simulink model "single_phase_ttype_inverter"  (R2026a)
settings: Solver=ode23tb  StopTime=simlength  FixedStep=tc  MaxStep=glb_time.tc
values from neighbouring files (symbols this model uses):
  afe_ctrl = param.afe.ctrl    [init_model.m]
  afe_pwm_phase_shift_mod1 = param.afe.behav.pwm_phase_shift_mod1    [init_model.m]
  DThs_init = param.thermal.DThs_init    [init_model.m]
  filters = param.ctrl.filters    [init_model.m]
  frt_data = param.frt.data    [init_model.m]
  glb_time = param.glb_time    [init_model.m]
  grid_emu = param.grid.emu    [init_model.m]
  kepsilon = param.spinv.kepsilon    [init_model.m]
  kp_align = param.ctrl.kp_align    [init_model.m]
  lim_down_align = param.ctrl.lim_down_align    [init_model.m]
  lim_up_align = param.ctrl.lim_up_align    [init_model.m]
  mavarage_filter_frequency_base_order = param.ctrl.mavarage_filter_frequency_base_order    [init_model.m]
  omega_set = param.spinv.omega_set    [init_model.m]
  single_phase_inverter_ctrl = param.spinv.ctrl    [init_model.m]
  Tambient = param.thermal.Tambient    [init_model.m]
  time_aux_power_supply_fault = param.sim.time_aux_power_supply_fault    [init_model.m]
  time_step_ref_1 = param.spinv.ref.time_step_ref_1    [init_model.m]
  time_step_ref_2 = param.spinv.ref.time_step_ref_2    [init_model.m]
  time_step_ref_3 = param.spinv.ref.time_step_ref_3    [init_model.m]
undefined symbols (not defined in the file or in its folder): delta_fht1, hwdata, ki_align, Ld_fht1, magnitude, omega_fht1, ts_inv, Vac_FS, Vdc_nom, Xbez
libraries: fl_lib x61, nesl_utility x39, moving_average_filter x11, moving_average_filter_cc x8, discrete_time_low_pass_filter x4, sl_discontinuities x3, single_phase_transformer_lib x3, linear_double_integrator_observer_ccaller x2, phase_shift_filter_ccaller x2, threephase_inductor_lib x1, dclink_for_two_levels x1, three_phase_pwm_modulator x1
(part 1 of 9)
settings Model: SimulationMode=accelerator  Creator=LTNBDA  LastModifiedBy=dbagn
settings SolverCC: ZeroCrossControl=EnableAll  ZeroCrossAlgorithm=Adaptive  SolverResetMethod=Robust
settings DataIOCC: MaxDataPoints=1  SignalLoggingSaveFormat=ModelDataLogs
settings OptimizationCC: InitFltsAndDblsToZero=on  EfficientMapNaN2IntZero=off
settings DebuggingCC: SaveWithParameterizedLinksMsg=none  UnderspecifiedInitializationDetection=Classic  SignalResolutionControl=TryResolveAllWithWarning  IgnoredZcDiagnostic=none  MultiTaskDSMMsg=warning  MultiTaskCondExecSysMsg=none  MultiTaskRateTransMsg=warning
settings HardwareCC: ProdBitPerLong=64.0  ProdHWDeviceType=Generic->64-bit Embedded Processor (LP64)  TargetBitPerPointer=64.0  TargetBitPerSizeT=64.0  TargetBitPerPtrDiffT=64.0  TargetLongLongMode=on  TargetIntDivRoundTo=Zero  TargetEndianess=LittleEndian  TargetWordSize=64.0  TargetHWDeviceType=MATLAB Host  ProdEqTarget=off
settings SFSimCC: SimCustomHeaderCode=|
  | #include "rpi.h"
  | #include "rpi_simulink.h"
  | #include "mavgflt.h"
  | #include "mavgflt_simulink.h"
  | #include "mavgflts.h"
  | #include "mavgflts_simulink.h"
  | #include "dsmavgflt.h"
  | #include "dsmavgflt_simulink.h"
  | #include "bemf_obsv.h"
  | #include "bemf_obsv_simulink.h"
  | #include "bemf_obsv_load_est.h"
  | #include "bemf_obsv_load_est_simulink.h"
  | #include "dqvector_pi.h"
  | #include "dqvector_pi_simulink.h"
  | #include "sv_pwm_simulink.h"
  | #include "sv_pwm.h"
  | #include "first_harmonic_tracker.h"
  | #include "first_harmonic_tracker_simulink.h"
  | #include "dqpll_thyr.h"
  | #include "dqpll_thyr_simulink.h"
  | #include "dqpll_grid.h"
  | #include "dqpll_grid_simulink.h"
  | #include "phase_shift_flt_simulink.h"
  | #include "phase_shift_flt.h"
  | #include "sogi_flt_simulink.h"
  | #include "sogi_flt.h"
  | #include "linear_double_integrator_observer_simulink.h"
  | #include "linear_double_integrator_observer.h"
settings SFSimCC: SimUserSources=|
  | "rpi.c"
  | "rpi_simulink.c"
  | "mavgflt_simulink.c"
  | "mavgflt.c"
  | "mavgflts_simulink.c"
  | "mavgflts.c"
  | "dsmavgflt_simulink.c"
  | "dsmavgflt.c"
  | "bemf_obsv_simulink.c"
  | "bemf_obsv.c"
  | "bemf_obsv_load_est_simulink.c"
  | "bemf_obsv_load_est.c"
  | "dqvector_pi.c"
  | "dqvector_pi_simulink.c"
  | "sv_pwm_simulink.c"
  | "sv_pwm.c"
  | "first_harmonic_tracker_simulink.c"
  | "first_harmonic_tracker.c"
  | "dqpll_thyr_simulink.c"
  | "dqpll_thyr.c"
  | "dqpll_grid_simulink.c"
  | "dqpll_grid.c"
  | "phase_shift_flt_simulink.c"
  | "phase_shift_flt.c"
  | "sogi_flt_simulink.c"
  | "sogi_flt.c"
  | "linear_double_integrator_observer_simulink.c"
  | "linear_double_integrator_observer.c"
settings SFSimCC: SimUserIncludeDirs=|
  | include
  | src
settings CodeAppCC: MaxIdLength=128.0
settings GRTTargetCC: CombineOutputUpdateFcns=off  GRTInterface=on
settings SimscapeCC: SimscapeNormalizeSystem=off  SimscapeNominalValues="[{\"value\":\"1\",\"unit\":\"A\"},{\"value\":\"1\",\"unit\":\"bar\"},{\"value\":\"1\",\"unit\":\"cm^2\"},{\"value\":\"1\",\"unit\":\"cm^3/s\"},{\"value\":\"1\",\"unit\":\"kJ/kg\"},{\"value\":\"1\",\"unit\":\"kW\"},{\"value\":\"1\",\"unit\":\"l\"},{\"value\":\"1\",\"unit\":\"N\"},{\"value\":\"1\",\"unit\":\"N*m\"},{\"value\":\"1\",\"unit\":\"V\"}]"  SimscapeLogType=none  SimscapeLogDataHistory=5000.0

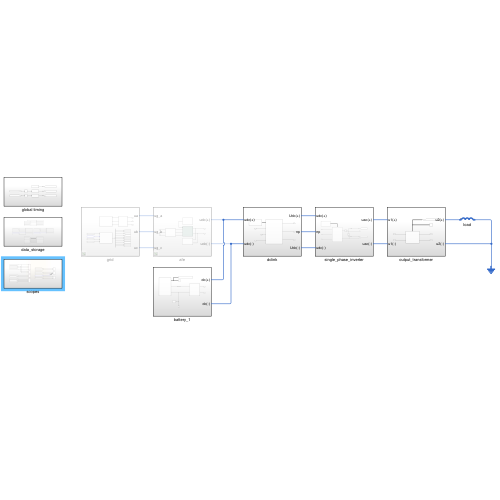
[thumbnail: Simulink's stored preview of the top-level diagram]
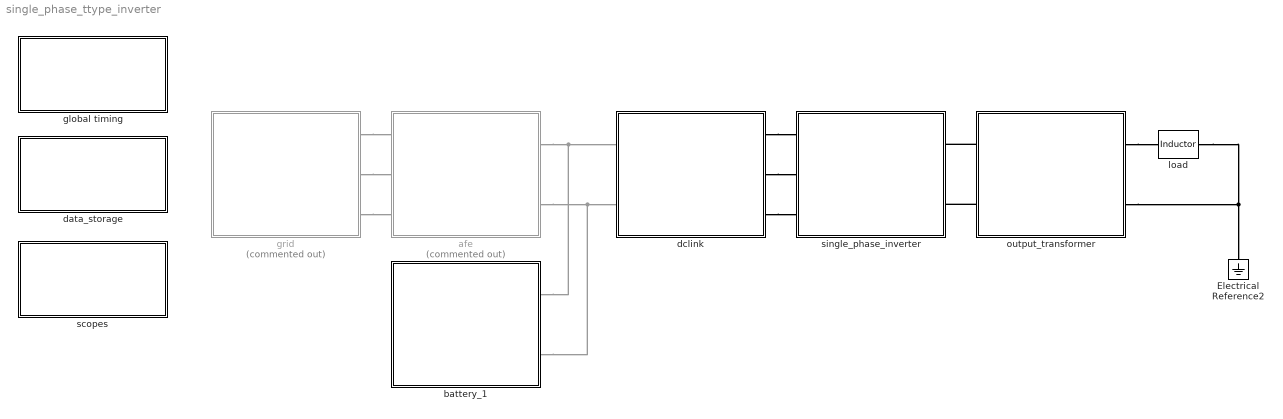
== system single_phase_ttype_inverter ==
  Electrical Reference2 : fl_lib/Electrical/Electrical Elements/Electrical Reference
  afe : Subsystem  Commented=on
  battery_1 : Subsystem
  data_storage : Subsystem
  dclink : Subsystem
  global timing : Subsystem
  grid : Subsystem  Commented=on
  load : fl_lib/Electrical/Electrical Elements/Inductor  l=lload H  r=rload Ohm  g=1e-9 1/Ohm  i_specify=off  i_priority=None  i=0 A  i_nominal_specify=off  i_nominal_value=1  i_nominal_unit=A  v_specify=off  v_priority=None  v=0 V  v_nominal_specify=off  v_nominal_value=1  v_nominal_unit=V  i_L_specify=off  i_L_priority=High  i_L=0 A  i_L_nominal_specify=off  i_L_nominal_value=1  i_L_nominal_unit=A
  output_transformer : Subsystem
  scopes : Subsystem
  single_phase_inverter : Subsystem
  connections:
  output_transformer/LConn1 -- single_phase_inverter/RConn1
  output_transformer/LConn2 -- single_phase_inverter/RConn2
  load/RConn1 -- output_transformer/RConn2 -- Electrical Reference2/LConn1
  output_transformer/RConn1 -- load/LConn1
  dclink/RConn1 -- single_phase_inverter/LConn1
  dclink/RConn2 -- single_phase_inverter/LConn2
  dclink/RConn3 -- single_phase_inverter/LConn3
  afe/RConn2 -- battery_1/RConn2 -- dclink/LConn2
  afe/RConn1 -- battery_1/RConn1 -- dclink/LConn1
  grid/RConn1 -- afe/LConn1
  grid/RConn2 -- afe/LConn2
  grid/RConn3 -- afe/LConn3

== system single_phase_ttype_inverter/afe ==
  AFE_control : Subsystem
  LCL_filter : Subsystem
  afe : Subsystem
  brake : Subsystem
  ug_a : PMIOPort  Side=Left
  udc(+) : PMIOPort  Port=2  Side=Right
  ug_b : PMIOPort  Port=3  Side=Left
  udc(-) : PMIOPort  Port=4  Side=Right
  ug_c : PMIOPort  Port=5  Side=Left
  wires:
  AFE_control/1(dabc_out) -> afe/1(dabc)
  connections:
  brake/LConn2 -- udc(-)/RConn1 -- afe/RConn2
  brake/LConn1 -- udc(+)/RConn1 -- afe/RConn1
  LCL_filter/LConn1 -- afe/LConn1
  LCL_filter/LConn2 -- afe/LConn2
  LCL_filter/LConn3 -- afe/LConn3
  ug_a/RConn1 -- LCL_filter/RConn1
  ug_b/RConn1 -- LCL_filter/RConn2
  ug_c/RConn1 -- LCL_filter/RConn3

== system single_phase_ttype_inverter/battery_1 ==
  Electrical Reference : fl_lib/Electrical/Electrical Elements/Electrical Reference
  Inductor : fl_lib/Electrical/Electrical Elements/Inductor  l=1e-3 H  r=0 Ohm  g=1e-9 1/Ohm  i_specify=off  i_priority=None  i=0 A  i_nominal_specify=off  i_nominal_value=1  i_nominal_unit=A  v_specify=off  v_priority=None  v=0 V  v_nominal_specify=off  v_nominal_value=1  v_nominal_unit=V  i_L_specify=off  i_L_priority=High  i_L=0 A  i_L_nominal_specify=off  i_L_nominal_value=1  i_L_nominal_unit=A
  Solver Configuration : nesl_utility/Solver Configuration  PhysicalDomain=network_engine_domain  SubClassName=solver  LeftPortType=input  RightPortType=generic  Tones=[]  Harmonics=[]  SimulateNoise=off  Profile=off  UseLocalSampling=off  EnableSwitchedLinearOptims=on  FrequencyDomain=off  UseCCode=off  RelTol=0.001  AbsTol=0.001  MinStep=1e-09  ToWorkspace=off  RevertToSquareIcSolve=off  NumHomotopyIterations=100  PhasorMode=off  PhasorModeNumHarmonics=1  ConsistencySolver=NEWTON_FTOL  CanonicalOrdering=UNORDERED  OptimizeIntermediates=UNOPTIMIZED  IndexReductionMethod=DerivativeReplacement  DoDC=on  ResidualTolerance=1e-3  ConsistencyTolSource=GLOBAL  ConsistencyAbsTol=0.001  ConsistencyRelTol=0.001  ConsistencyTolFactor=0.001  UseLocalSolver=on  LocalSolverChoice=NE_BACKWARD_EULER_ADVANCER  ResolveIndetEquations=on  FunctionEvalNumThread=1  LocalSolverSampleTime=glb_time.tc  DoFixedCost=on  MaxNonlinIter=nonlinear_iterations  MaxModeIter=2  ComputeImpulses=off  ImpulseIterations=2  LinearAlgebra=auto  LinearAlgebraNumThread=0  EquationFormulation=NE_TIME_EF  DelaysMemoryBudget=1024  AutomaticFiltering=on  FilteringTimeConstant=0.001  PartitionStorageMethod=AS_NEEDED  PartitionMemoryBudget=1024  PartitionMethod=ROBUST  MultibodyUseLocalSolver=off  MultibodyLocalSolverChoice=ODE1  MultibodyLocalSolverSampleTime=0.001
  To Workspace14 : ToWorkspace  VariableName=battery_1_data_sim  SampleTime=glb_time.tc
      settings: MaxDataPoints=glb_time.Nc  Decimation=glb_time.decimation_tc
  lithium ion battery : Scope
      settings: ActiveDisplayYMinimum=-808.27997881012811  ActiveDisplayYMaximum=1287.7546757937268  DataLoggingVariableName=ScopeData3
  lithium_ion_battery : lithium_ion_battery/lithium_ion_battery  Q=lithium_ion_battery_1.Q  number_of_cells=lithium_ion_battery_1.number_of_cells  E_1=lithium_ion_battery_1.E_1  E0=lithium_ion_battery_1.E0  E1=lithium_ion_battery_1.E1  E2=lithium_ion_battery_1.E2  E3=lithium_ion_battery_1.E3  Elog=lithium_ion_battery_1.Elog  R0=lithium_ion_battery_1.R0  R1=lithium_ion_battery_1.R1  C1=lithium_ion_battery_1.C1  M=lithium_ion_battery_1.M  alpha=lithium_ion_battery_1.alpha  soc_init=lithium_ion_battery_1.soc_init  ts_battery=glb_time.ts_dab  q1Kalman=lithium_ion_battery_1.q1Kalman  q2Kalman=lithium_ion_battery_1.q2Kalman  q3Kalman=lithium_ion_battery_1.q3Kalman  rKalman=lithium_ion_battery_1.rKalman  tc=glb_time.tc  enable_white_noise_m=0
  single_phase_ui_measure : Subsystem
  dc(+) : PMIOPort  Side=Right
  dc(-) : PMIOPort  Port=2  Side=Right
  wires:
  lithium_ion_battery/1 -> To Workspace14/1, lithium ion battery/1
  connections:
  lithium_ion_battery/RConn2 -- single_phase_ui_measure/LConn2 -- Solver Configuration/RConn1 -- Electrical Reference/LConn1
  single_phase_ui_measure/RConn1 -- dc(+)/RConn1
  Inductor/LConn1 -- lithium_ion_battery/RConn1
  dc(-)/RConn1 -- single_phase_ui_measure/RConn2
  single_phase_ui_measure/LConn1 -- Inductor/RConn1

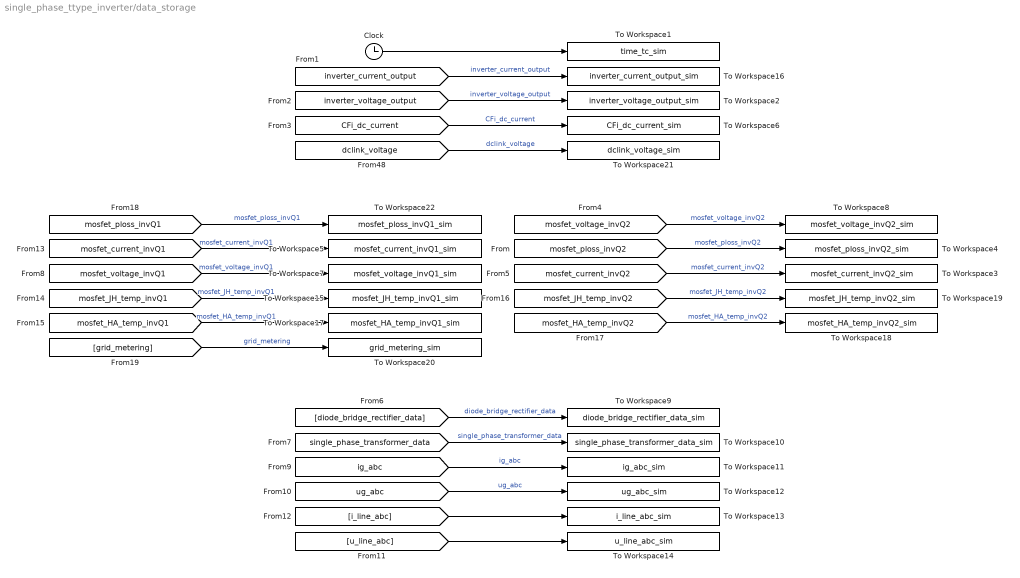
== system single_phase_ttype_inverter/data_storage ==
  Clock : Clock
  To Workspace1 : ToWorkspace  VariableName=time_tc_sim  SampleTime=glb_time.tc
      settings: MaxDataPoints=glb_time.Nc  Decimation=glb_time.decimation_tc
  To Workspace10 : ToWorkspace  VariableName=single_phase_transformer_data_sim  SampleTime=glb_time.tc
      settings: MaxDataPoints=glb_time.Nc  Decimation=glb_time.decimation_tc
  To Workspace11 : ToWorkspace  VariableName=ig_abc_sim  SampleTime=glb_time.tc
      settings: MaxDataPoints=glb_time.Nc  Decimation=glb_time.decimation_tc
  To Workspace12 : ToWorkspace  VariableName=ug_abc_sim  SampleTime=glb_time.tc
      settings: MaxDataPoints=glb_time.Nc  Decimation=glb_time.decimation_tc
  To Workspace13 : ToWorkspace  VariableName=i_line_abc_sim  SampleTime=glb_time.tc
      settings: MaxDataPoints=glb_time.Nc  Decimation=glb_time.decimation_tc
  To Workspace14 : ToWorkspace  VariableName=u_line_abc_sim  SampleTime=glb_time.tc
      settings: MaxDataPoints=glb_time.Nc  Decimation=glb_time.decimation_tc
  To Workspace15 : ToWorkspace  VariableName=mosfet_JH_temp_invQ1_sim  SampleTime=glb_time.tc
      settings: MaxDataPoints=glb_time.Nc  Decimation=glb_time.decimation_tc
  To Workspace16 : ToWorkspace  VariableName=inverter_current_output_sim  SampleTime=glb_time.tc
      settings: MaxDataPoints=glb_time.Nc  Decimation=glb_time.decimation_tc
  To Workspace17 : ToWorkspace  VariableName=mosfet_HA_temp_invQ1_sim  SampleTime=glb_time.tc
      settings: MaxDataPoints=glb_time.Nc  Decimation=glb_time.decimation_tc
  To Workspace18 : ToWorkspace  VariableName=mosfet_HA_temp_invQ2_sim  SampleTime=glb_time.tc
      settings: MaxDataPoints=glb_time.Nc  Decimation=glb_time.decimation_tc
  To Workspace19 : ToWorkspace  VariableName=mosfet_JH_temp_invQ2_sim  SampleTime=glb_time.tc
      settings: MaxDataPoints=glb_time.Nc  Decimation=glb_time.decimation_tc
  To Workspace2 : ToWorkspace  VariableName=inverter_voltage_output_sim  SampleTime=glb_time.tc
      settings: MaxDataPoints=glb_time.Nc  Decimation=glb_time.decimation_tc
  To Workspace20 : ToWorkspace  VariableName=grid_metering_sim  SampleTime=glb_time.tc
      settings: MaxDataPoints=glb_time.Nc  Decimation=glb_time.decimation_tc
  To Workspace21 : ToWorkspace  VariableName=dclink_voltage_sim  SampleTime=glb_time.tc
      settings: MaxDataPoints=glb_time.Nc  Decimation=glb_time.decimation_tc
  To Workspace22 : ToWorkspace  VariableName=mosfet_ploss_invQ1_sim  SampleTime=glb_time.tc
      settings: MaxDataPoints=glb_time.Nc  Decimation=glb_time.decimation_tc
  To Workspace3 : ToWorkspace  VariableName=mosfet_current_invQ2_sim  SampleTime=glb_time.tc
      settings: MaxDataPoints=glb_time.Nc  Decimation=glb_time.decimation_tc
  To Workspace4 : ToWorkspace  VariableName=mosfet_ploss_invQ2_sim  SampleTime=glb_time.tc
      settings: MaxDataPoints=glb_time.Nc  Decimation=glb_time.decimation_tc
  To Workspace5 : ToWorkspace  VariableName=mosfet_current_invQ1_sim  SampleTime=glb_time.tc
      settings: MaxDataPoints=glb_time.Nc  Decimation=glb_time.decimation_tc
  To Workspace6 : ToWorkspace  VariableName=CFi_dc_current_sim  SampleTime=glb_time.tc
      settings: MaxDataPoints=glb_time.Nc  Decimation=glb_time.decimation_tc
  To Workspace7 : ToWorkspace  VariableName=mosfet_voltage_invQ1_sim  SampleTime=glb_time.tc
      settings: MaxDataPoints=glb_time.Nc  Decimation=glb_time.decimation_tc
  To Workspace8 : ToWorkspace  VariableName=mosfet_voltage_invQ2_sim  SampleTime=glb_time.tc
      settings: MaxDataPoints=glb_time.Nc  Decimation=glb_time.decimation_tc
  To Workspace9 : ToWorkspace  VariableName=diode_bridge_rectifier_data_sim  SampleTime=glb_time.tc
      settings: MaxDataPoints=glb_time.Nc  Decimation=glb_time.decimation_tc
  wires:
  Clock/1 -> To Workspace1/1
  [inverter_current_output] -> To Workspace16/1  "inverter_current_output"
  [inverter_voltage_output] -> To Workspace2/1  "inverter_voltage_output"
  [CFi_dc_current] -> To Workspace6/1  "CFi_dc_current"
  [mosfet_ploss_invQ1] -> To Workspace22/1  "mosfet_ploss_invQ1"
  [dclink_voltage] -> To Workspace21/1  "dclink_voltage"
  [mosfet_current_invQ1] -> To Workspace5/1  "mosfet_current_invQ1"
  [mosfet_current_invQ2] -> To Workspace3/1  "mosfet_current_invQ2"
  [mosfet_ploss_invQ2] -> To Workspace4/1  "mosfet_ploss_invQ2"
  [mosfet_voltage_invQ1] -> To Workspace7/1  "mosfet_voltage_invQ1"
  [mosfet_voltage_invQ2] -> To Workspace8/1  "mosfet_voltage_invQ2"
  [diode_bridge_rectifier_data] -> To Workspace9/1  "diode_bridge_rectifier_data"
  [single_phase_transformer_data] -> To Workspace10/1  "single_phase_transformer_data"
  [ig_abc] -> To Workspace11/1  "ig_abc"
  [ug_abc] -> To Workspace12/1  "ug_abc"
  [i_line_abc] -> To Workspace13/1
  [u_line_abc] -> To Workspace14/1
  [mosfet_JH_temp_invQ1] -> To Workspace15/1  "mosfet_JH_temp_invQ1"
  [mosfet_HA_temp_invQ1] -> To Workspace17/1  "mosfet_HA_temp_invQ1"
  [mosfet_JH_temp_invQ2] -> To Workspace19/1  "mosfet_JH_temp_invQ2"
  [mosfet_HA_temp_invQ2] -> To Workspace18/1  "mosfet_HA_temp_invQ2"
  [grid_metering] -> To Workspace20/1  "grid_metering"

== system single_phase_ttype_inverter/dclink ==
  Open Circuit : fl_lib/Electrical/Electrical Elements/Open Circuit  v_specify=off  v_priority=None  v=0 V  v_nominal_specify=off  v_nominal_value=1  v_nominal_unit=V
  dclink : dclink_for_three_levels/dclink  Cdc1_m=hwdata.single_phase_inverter.CFi1  Cdc2_m=hwdata.single_phase_inverter.CFi2  Rudc_measure=107e3  Vdc_scale=hwdata.single_phase_inverter.udc_nom  Vdc1_m_init=hwdata.single_phase_inverter.udc_nom/2  Vdc2_m_init=hwdata.single_phase_inverter.udc_nom/2
  references : Subsystem
  Udc(+) : PMIOPort  Side=Right
  np : PMIOPort  Port=2  Side=Right
  Udc(-) : PMIOPort  Port=3  Side=Right
  udc(+) : PMIOPort  Port=4  Side=Left
  udc(-) : PMIOPort  Port=5  Side=Left
  wires:
  dclink/1 -> references/1(m)
  connections:
  Open Circuit/LConn1 -- dclink/RConn2
  udc(+)/RConn1 -- dclink/RConn1
  udc(-)/RConn1 -- dclink/RConn3
  Udc(+)/RConn1 -- dclink/LConn1
  Udc(-)/RConn1 -- dclink/LConn3
  dclink/LConn2 -- np/RConn1

== system single_phase_ttype_inverter/global timing ==
  Unit Delay : UnitDelay  SampleTime=glb_time.tc
  Unit Delay1 : UnitDelay  SampleTime=glb_time.tc
  time_afe1 : Subsystem  mask{k=1}
      mask prompts: k "Time Gain"
      mask Display:
      | disp('time-gen');
      | port_label('input', 1, 'crt');
      | port_label('output', 1, 'tout');
  time_afe2 : Subsystem  mask{k=1}
      mask prompts: k "Time Gain"
      mask Display:
      | disp('time-gen');
      | port_label('input', 1, 'crt');
      | port_label('output', 1, 'tout');
  time_afe3 : Subsystem  mask{k=1}
      mask prompts: k "Time Gain"
      mask Display:
      | disp('time-gen');
      | port_label('output', 1, 'tout');
  tag scope: local_time_afe=global, local_time_inverter=global, time_master=global
  wires:
  time_afe1/1(Out1) -> [local_time_afe]
  time_afe3/1(Out1) -> [time_master]
  [local_time_corr_afe] -> Unit Delay/1
  Unit Delay/1 -> time_afe1/1(correction_time)
  Unit Delay1/1 -> time_afe2/1(correction_time)
  [local_time_corr_inv] -> Unit Delay1/1
  time_afe2/1(Out1) -> [local_time_inverter]

== system single_phase_ttype_inverter/grid ==
  Bus Selector : BusSelector  OutputSignals=Q1p,Q1n,P1n,P1p,U1n,U1p,i_act_1n,i_react_1n,i_act_1p,i_react_1p
  To Workspace1 : ToWorkspace  VariableName=i_react_1n  SampleTime=glb_time.ts_afe
      settings: MaxDataPoints=glb_time.Ns_afe
  To Workspace2 : ToWorkspace  VariableName=i_react_1p  SampleTime=glb_time.ts_afe
      settings: MaxDataPoints=glb_time.Ns_afe
  To Workspace3 : ToWorkspace  VariableName=i_act_1n  SampleTime=glb_time.ts_afe
      settings: MaxDataPoints=glb_time.Ns_afe
  To Workspace4 : ToWorkspace  VariableName=i_act_1p  SampleTime=glb_time.ts_afe
      settings: MaxDataPoints=glb_time.Ns_afe
  To Workspace5 : ToWorkspace  VariableName=u1p  SampleTime=glb_time.ts_afe
      settings: MaxDataPoints=glb_time.Ns_afe
  To Workspace6 : ToWorkspace  VariableName=u1n  SampleTime=glb_time.ts_afe
      settings: MaxDataPoints=glb_time.Ns_afe
  grid_emulator : Subsystem
  power meter iec : power_meter_iec/power meter iec  period=pi/grid_emu.omega_grid_nom  ts=glb_time.ts_afe  enable_time=0.025
  threephase_vi_measures : Subsystem
  ua : PMIOPort  Side=Right
  ub : PMIOPort  Port=2  Side=Right
  uc : PMIOPort  Port=3  Side=Right
  tag scope: P1n_global=global, P1p_global=global, Q1n_global=global, Q1p_global=global
  wires:
  [gamma_grid_emulator] -> power meter iec/1
  [ug_abc] -> power meter iec/2
  [ig_abc] -> power meter iec/3
  power meter iec/1 -> Bus Selector/1
  Bus Selector/1 -> [Q1p_global]  "<Q1p>"
  Bus Selector/2 -> [Q1n_global]  "<Q1n>"
  Bus Selector/3 -> [P1n_global]  "<P1n>"
  Bus Selector/4 -> [P1p_global]  "<P1p>"
  Bus Selector/5 -> To Workspace6/1  "<U1n>"
  Bus Selector/6 -> To Workspace5/1  "<U1p>"
  Bus Selector/7 -> To Workspace3/1  "<i_act_1n>"
  Bus Selector/8 -> To Workspace1/1  "<i_react_1n>"
  Bus Selector/9 -> To Workspace4/1  "<i_act_1p>"
  Bus Selector/10 -> To Workspace2/1  "<i_react_1p>"
  [omega_grid_emulator] -> power meter iec/4
  connections:
  threephase_vi_measures/LConn3 -- grid_emulator/RConn3
  threephase_vi_measures/LConn1 -- grid_emulator/RConn1
  threephase_vi_measures/RConn2 -- ub/RConn1
  threephase_vi_measures/LConn2 -- grid_emulator/RConn2
  threephase_vi_measures/RConn1 -- ua/RConn1
  threephase_vi_measures/RConn3 -- uc/RConn1

== system single_phase_ttype_inverter/output_transformer ==
  single_phase_transformer : single_phase_transformer/single_phase_transformer  lm_trafo=output_transformer.Lm1  m1=output_transformer.n1  m2=output_transformer.n2  rd1_trafo=output_transformer.Rd1  rd2_trafo=output_transformer.Rd2  ld1_trafo=output_transformer.Ld1  ld2_trafo=output_transformer.Ld2  rfe_trafo=output_transformer.Rfe1  length_core=1  mu0=1.256637e-6  mur=2200
  single_phase_transformer - scope : Scope
      settings: ActiveDisplayYMinimum=1.9526662119496512  ActiveDisplayYMaximum=2.25212456388615  DataLoggingVariableName=ScopeData11
  u1(+) : PMIOPort  Side=Left
  u2(+) : PMIOPort  Port=2  Side=Right
  u1(-) : PMIOPort  Port=3  Side=Left
  u2(-) : PMIOPort  Port=4  Side=Right
  tag scope: single_phase_transformer_data=global
  wires:
  single_phase_transformer/1 -> [single_phase_transformer_data], single_phase_transformer - scope/1
  connections:
  single_phase_transformer/LConn2 -- u1(-)/RConn1
  single_phase_transformer/LConn1 -- u1(+)/RConn1
  single_phase_transformer/RConn1 -- u2(+)/RConn1
  single_phase_transformer/RConn2 -- u2(-)/RConn1

== system single_phase_ttype_inverter/scopes ==
  Bus Creator : BusCreator  Inputs=2
  dclink voltage : Scope  NumInputPorts=3
      settings: SampleTime=glb_time.tc  ActiveDisplayString=3  ActiveDisplayYMinimum=-1  ActiveDisplayYMaximum=1  DataLoggingVariableName=ScopeData9
  ig_abc/ug_abc : Scope  NumInputPorts=2
      settings: SampleTime=glb_time.tc  ActiveDisplayYMinimum=-478.59349677124044  ActiveDisplayYMaximum=478.39144343621263  DataLoggingVariableName=ScopeData5
  inverter current/voltage : Scope  NumInputPorts=4
      settings: ActiveDisplayYMinimum=-1104.7741618114699  ActiveDisplayYMaximum=1101.5054352731458
  inverter current/voltage output : Scope  NumInputPorts=2
      settings: ActiveDisplayYMinimum=-1760.965659691359  ActiveDisplayYMaximum=1772.299605358274
  iu-mosfet-invQ1 : Scope  NumInputPorts=2
      settings: SampleTime=glb_time.tc  ActiveDisplayYMinimum=-1884.5917198054758  ActiveDisplayYMaximum=2532.7760155502147  DataLoggingVariableName=ScopeData7
  power_loss mosfet_inv : Scope  NumInputPorts=2
      settings: SampleTime=glb_time.tc  ActiveDisplayYMinimum=-56.04719512944142  ActiveDisplayYMaximum=547.23959786612  DataLoggingVariableName=ScopeData6
  udc 1&2 : Scope  NumInputPorts=2
      settings: SampleTime=glb_time.tc  ActiveDisplayYMinimum=623.18302864677787  ActiveDisplayYMaximum=624.17967210308166  DataLoggingVariableName=ScopeData4
  wires:
  [idc1_m] -> inverter current/voltage/3  "idc1_m"
  [inverter_voltage_output] -> inverter current/voltage/2, inverter current/voltage output/1  "inverter_voltage_output_modA"
  [inverter_current_output] -> inverter current/voltage/1, inverter current/voltage output/2  "inverter_current_output_modA"
  [idc2_m] -> inverter current/voltage/4  "idc2_m"
  [udc1_m] -> udc 1&2/1  "udc1_m"
  [udc2_m] -> udc 1&2/2  "udc2_m"
  [ug_abc] -> ig_abc/ug_abc/2  "vg_abc"
  [ig_abc] -> ig_abc/ug_abc/1  "ig_abc"
  [mosfet_ploss_invQ1] -> power_loss mosfet_inv/1  "mosfet_ploss_invQ1"
  [mosfet_JH_temp_invQ1] -> Bus Creator/1  "mosfet_JH_temp_invQ1"
  [mosfet_HA_temp_invQ1] -> Bus Creator/2  "mosfet_HA_temp_invQ1"
  Bus Creator/1 -> power_loss mosfet_inv/2
  [mosfet_current_invQ1] -> iu-mosfet-invQ1/1  "mosfet_current_invQ1"
  [mosfet_voltage_invQ1] -> iu-mosfet-invQ1/2  "mosfet_voltage_invQ1"
  [dclink_voltage] -> dclink voltage/1  "dclink_voltage"
  [dclink_p2gnd_voltage] -> dclink voltage/2  "dclink_p2gnd_voltage"
  [dclink_n2gnd_voltage] -> dclink voltage/3  "dclink_n2gnd_voltage"

== system single_phase_ttype_inverter/single_phase_inverter ==
  Current Sensor : fl_lib/Electrical/Electrical Sensors/Current Sensor
  Voltage Sensor1 : fl_lib/Electrical/Electrical Sensors/Voltage Sensor
  iph : nesl_utility/PS-Simulink Converter  PhysicalDomain=network_engine_domain  SubClassName=ps_output  LeftPortType=input  RightPortType=output  PseudoPeriodic=off  Frequencies=[]  VectorFormat=1-D array  Unit=A  AffineConversion=off
  single phase inverter : Subsystem
      settings: PortSchema="{\"entries\":[{\"content\":{\"sides\":[{\"content\":{\"connectorIds\":[\"LConn1\",\"LConn2\"]},\"type\":\"ConnectorPlacement.EquallySpacedRectSide\",\"uuid\":\"4fcf4fea-d38f-431b-8a91-be3ce9782faf\"},{\"content\":{\"connectorIds\":[\"RConn1\",\"RConn2\",\"RConn3\"],\"side\":\"RIGHT\"},\"type\":\"ConnectorPlacement.EquallySpacedRectSide\",\"uuid\":\"0aa56277-92e9-4e3b-84c7-43398254a4d8\"},{\"content\":{\"connectorIds\":[\"In1\"],\"side\":\"TOP\"},\"type\":\"ConnectorPlacement.EquallySpacedRectSide\",\"uuid\":\"5cd150dc-bcaf-4cd7-b2a8-3db203726730\"}]},\"type\":\"ConnectorPlacement.EquallySpacedConnector\",\"uuid\":\"bf8194c4-c327-4d40-bea4-f1e7617f80b4\"}],\"packageUris\":[\"http://schema.mathworks.com/mf0/Connector/R2020b\"],\"version\":\"1.0\"}"
  single phase inverter control : Subsystem
  uph1 : nesl_utility/PS-Simulink Converter  PhysicalDomain=network_engine_domain  SubClassName=ps_output  LeftPortType=input  RightPortType=output  PseudoPeriodic=off  Frequencies=[]  VectorFormat=1-D array  Unit=V  AffineConversion=off
  uac(+) : PMIOPort  Side=Right
  uac(-) : PMIOPort  Port=2  Side=Right
  udc(+) : PMIOPort  Port=3  Side=Left
  np : PMIOPort  Port=4  Side=Left
  udc(-) : PMIOPort  Port=5  Side=Left
  tag scope: inverter_current_output=global, inverter_voltage_output=global
  wires:
  single phase inverter control/1(gate_cmds) -> single phase inverter/1(gate_commands)
  iph/1 -> [inverter_current_output]  "inverter_current_output"
  uph1/1 -> [inverter_voltage_output]  "inverter_voltage_output"
  connections:
  single phase inverter/LConn1 -- Current Sensor/LConn1
  uac(-)/RConn1 -- single phase inverter/LConn2 -- Voltage Sensor1/RConn2
  Voltage Sensor1/RConn1 -- uph1/LConn1
  iph/LConn1 -- Current Sensor/RConn1
  uac(+)/RConn1 -- Current Sensor/RConn2 -- Voltage Sensor1/LConn1
  single phase inverter/RConn1 -- udc(+)/RConn1
  single phase inverter/RConn3 -- udc(-)/RConn1
  np/RConn1 -- single phase inverter/RConn2

== system single_phase_ttype_inverter/afe/AFE_control ==
  afe_control : Subsystem
  dabc_out : Outport
  tag scope: local_time_corr_afe=global
  wires:
  [TRGO_afe_module_1] -> afe_control/Trigger
  [ug_abc_pu_mod1] -> afe_control/1(ug_abc_pu)
  [is_abc_pu_mod1] -> afe_control/4(is_abc_pu)
  [vdc_pu_afe_mod1] -> afe_control/2(udc_pu)
  afe_control/1(duvw) -> dabc_out/1
  [ig_abc_pu_mod1] -> afe_control/3(ig_abc_pu)
  [local_time_afe] -> afe_control/5(local_time)
  [time_master] -> afe_control/6(master_time)
  afe_control/2(AFE1_local_time_corr) -> [local_time_corr_afe]
  [gamma_grid_emulator] -> afe_control/7(grid_phase)

== system single_phase_ttype_inverter/afe/LCL_filter ==
  CFu1 : fl_lib/Electrical/Electrical Elements/Capacitor  c=hwdata.afe.CFu F  r=hwdata.afe.RCFu Ohm  g=0 1/Ohm  i_specify=off  i_priority=None  i=0 A  i_nominal_specify=off  i_nominal_value=1  i_nominal_unit=A  v_specify=off  v_priority=None  v=0 V  v_nominal_specify=off  v_nominal_value=1  v_nominal_unit=V  vc_specify=off  vc_priority=High  vc=0 V  vc_nominal_specify=off  vc_nominal_value=1  vc_nominal_unit=V
  CFu2 : fl_lib/Electrical/Electrical Elements/Capacitor  c=hwdata.afe.CFu F  r=hwdata.afe.RCFu Ohm  g=0 1/Ohm  i_specify=off  i_priority=None  i=0 A  i_nominal_specify=off  i_nominal_value=1  i_nominal_unit=A  v_specify=off  v_priority=None  v=0 V  v_nominal_specify=off  v_nominal_value=1  v_nominal_unit=V  vc_specify=off  vc_priority=High  vc=0 V  vc_nominal_specify=off  vc_nominal_value=1  vc_nominal_unit=V
  CFu3 : fl_lib/Electrical/Electrical Elements/Capacitor  c=hwdata.afe.CFu F  r=hwdata.afe.RCFu Ohm  g=0 1/Ohm  i_specify=off  i_priority=None  i=0 A  i_nominal_specify=off  i_nominal_value=1  i_nominal_unit=A  v_specify=off  v_priority=None  v=0 V  v_nominal_specify=off  v_nominal_value=1  v_nominal_unit=V  vc_specify=off  vc_priority=High  vc=0 V  vc_nominal_specify=off  vc_nominal_value=1  vc_nominal_unit=V
  Inductor : fl_lib/Electrical/Electrical Elements/Inductor  l=1e-6 H  r=0 Ohm  g=1e-9 1/Ohm  i_specify=on  i_priority=High  i=0 A  i_nominal_specify=off  i_nominal_value=1  i_nominal_unit=A  v_specify=off  v_priority=None  v=0 V  v_nominal_specify=off  v_nominal_value=1  v_nominal_unit=V  i_L_specify=off  i_L_priority=High  i_L=0 A  i_L_nominal_specify=off  i_L_nominal_value=1  i_L_nominal_unit=A
  Inductor1 : fl_lib/Electrical/Electrical Elements/Inductor  l=1e-6 H  r=0 Ohm  g=1e-9 1/Ohm  i_specify=on  i_priority=High  i=0 A  i_nominal_specify=off  i_nominal_value=1  i_nominal_unit=A  v_specify=off  v_priority=None  v=0 V  v_nominal_specify=off  v_nominal_value=1  v_nominal_unit=V  i_L_specify=off  i_L_priority=High  i_L=0 A  i_L_nominal_specify=off  i_L_nominal_value=1  i_L_nominal_unit=A
  Inductor2 : fl_lib/Electrical/Electrical Elements/Inductor  l=1e-6 H  r=0 Ohm  g=1e-9 1/Ohm  i_specify=on  i_priority=High  i=0 A  i_nominal_specify=off  i_nominal_value=1  i_nominal_unit=A  v_specify=off  v_priority=None  v=0 V  v_nominal_specify=off  v_nominal_value=1  v_nominal_unit=V  i_L_specify=off  i_L_priority=High  i_L=0 A  i_L_nominal_specify=off  i_L_nominal_value=1  i_L_nominal_unit=A
  threephase inductor : threephase_inductor_lib/threephase inductor  Lp=hwdata.afe.LFu H  L0=hwdata.afe.LFu_cm H  Rp=hwdata.afe.RLFu Ohm  R0=hwdata.afe.RLFu_cm Ohm  Lls=5e-6 H  uu_1_specify=off  uu_1_priority=None  uu_1=0 V  uu_1_nominal_specify=off  uu_1_nominal_value=1  uu_1_nominal_unit=V  uv_1_specify=off  uv_1_priority=None  uv_1=0 V  uv_1_nominal_specify=off  uv_1_nominal_value=1  uv_1_nominal_unit=V  uw_1_specify=off  uw_1_priority=None  uw_1=0 V  uw_1_nominal_specify=off  uw_1_nominal_value=1  uw_1_nominal_unit=V  uu_2_specify=off  uu_2_priority=None  uu_2=0 V  uu_2_nominal_specify=off  uu_2_nominal_value=1  uu_2_nominal_unit=V  uv_2_specify=off  uv_2_priority=None  uv_2=0 V  uv_2_nominal_specify=off  uv_2_nominal_value=1  uv_2_nominal_unit=V  uw_2_specify=off  uw_2_priority=None  uw_2=0 V  uw_2_nominal_specify=off  uw_2_nominal_value=1  uw_2_nominal_unit=V  iu_specify=off  iu_priority=High  iu=0 A  iu_nominal_specify=off  iu_nominal_value=1  iu_nominal_unit=A  iv_specify=off  iv_priority=High  iv=0 A  iv_nominal_specify=off  iv_nominal_value=1  iv_nominal_unit=A  iw_specify=off  iw_priority=High  iw=0 A  iw_nominal_specify=off  iw_nominal_value=1  iw_nominal_unit=A
  threephase_vi_measures_stack : Subsystem
  threephase_vi_measures_stack1 : Subsystem
  us_a : PMIOPort  Side=Left
  ug_a : PMIOPort  Port=2  Side=Right
  us_b : PMIOPort  Port=3  Side=Left
  ug_b : PMIOPort  Port=4  Side=Right
  us_c : PMIOPort  Port=5  Side=Left
  ug_c : PMIOPort  Port=6  Side=Right
  connections:
  CFu1/RConn1 -- CFu3/RConn1 -- CFu2/RConn1
  Inductor/RConn1 -- threephase_vi_measures_stack1/LConn1 -- CFu1/LConn1
  Inductor2/RConn1 -- CFu3/LConn1 -- threephase_vi_measures_stack1/LConn3
  Inductor1/RConn1 -- CFu2/LConn1 -- threephase_vi_measures_stack1/LConn2
  threephase_vi_measures_stack/LConn1 -- us_a/RConn1
  threephase_vi_measures_stack/LConn2 -- us_b/RConn1
  threephase_vi_measures_stack/LConn3 -- us_c/RConn1
  threephase_vi_measures_stack/RConn1 -- threephase inductor/LConn1
  threephase_vi_measures_stack/RConn2 -- threephase inductor/LConn2
  threephase_vi_measures_stack/RConn3 -- threephase inductor/LConn3
  threephase inductor/RConn1 -- Inductor/LConn1
  Inductor1/LConn1 -- threephase inductor/RConn2
  Inductor2/LConn1 -- threephase inductor/RConn3
  ug_a/RConn1 -- threephase_vi_measures_stack1/RConn1
  ug_b/RConn1 -- threephase_vi_measures_stack1/RConn2
  ug_c/RConn1 -- threephase_vi_measures_stack1/RConn3

== system single_phase_ttype_inverter/afe/afe ==
  dabc : Inport
  Bus Selector : BusSelector  OutputSignals=vdc_pu
  Bus Selector1 : BusSelector  OutputSignals=udc,udc_p_gnd,udc_centertap_gnd,udc_n_gnd  OutputAsBus=on
  Bus Selector2 : BusSelector  OutputSignals=udc
  Bus Selector3 : BusSelector  OutputSignals=Cdc1_current
  dclink1 : dclink_for_two_levels/dclink  Cdc=hwdata.afe.CFi  Rudc_measure=1e6  Vdc_scale=hwdata.afe.udc_nom
  sv_pwm : Subsystem
  three_phase_inverter_ideal_switch_based_model : three_phase_inverter_ideal_switch_based_model/three phase inverter ideal switch based model  Ron_ideal_switch=ideal_switch.Rds_on  Vth=ideal_switch.Vth  Vgamma=ideal_switch.Vdon_diode  Rdon_diode=ideal_switch.Rdon_diode  Csnubber=ideal_switch.Csnubber  Rsnubber=ideal_switch.Rsnubber
  three_phase_inverter_igbt_based_with_thermal_model : Subsystem  Commented=on
  three_phase_inverter_mosfet_based_with_thermal_model : Subsystem  Commented=on
  us_a : PMIOPort  Side=Left
  us_b : PMIOPort  Port=2  Side=Left
  us_c : PMIOPort  Port=3  Side=Left
  Udc(+) : PMIOPort  Port=4  Side=Right
  Udc(-) : PMIOPort  Port=5  Side=Right
  tag scope: all_voltages_about_dclink=global, ic_dclink_mod1=global, udc_mod1=global, vdc_pu_afe_mod1=global, vdc_pu_inv_mod1=global
  wires:
  dabc/1 -> sv_pwm/1(duties_uvw)
  sv_pwm/1(gate_cmds) -> three_phase_inverter_mosfet_based_with_thermal_model/1(gate_commands), three_phase_inverter_igbt_based_with_thermal_model/1(gate_commands), three_phase_inverter_ideal_switch_based_model/1
  dclink1/1 -> Bus Selector1/1, Bus Selector2/1, Bus Selector3/1, Bus Selector/1
  Bus Selector1/1 -> [all_voltages_about_dclink]
  Bus Selector/1 -> [vdc_pu_afe_mod1], [vdc_pu_inv_mod1]  "<vdc_pu>"
  Bus Selector2/1 -> [udc_mod1]  "<udc>"
  Bus Selector3/1 -> [ic_dclink_mod1]  "<Cdc1_current>"
  connections:
  us_b/RConn1 -- three_phase_inverter_mosfet_based_with_thermal_model/RConn2 -- three_phase_inverter_ideal_switch_based_model/RConn2 -- three_phase_inverter_igbt_based_with_thermal_model/RConn2
  dclink1/RConn1 -- Udc(+)/RConn1
  dclink1/RConn2 -- Udc(-)/RConn1
  three_phase_inverter_igbt_based_with_thermal_model/RConn1 -- three_phase_inverter_mosfet_based_with_thermal_model/RConn1 -- three_phase_inverter_ideal_switch_based_model/RConn1 -- us_a/RConn1
  us_c/RConn1 -- three_phase_inverter_mosfet_based_with_thermal_model/RConn3 -- three_phase_inverter_ideal_switch_based_model/RConn3 -- three_phase_inverter_igbt_based_with_thermal_model/RConn3
  dclink1/LConn2 -- three_phase_inverter_ideal_switch_based_model/LConn2 -- three_phase_inverter_igbt_based_with_thermal_model/LConn2 -- three_phase_inverter_mosfet_based_with_thermal_model/LConn2
  dclink1/LConn1 -- three_phase_inverter_ideal_switch_based_model/LConn1 -- three_phase_inverter_igbt_based_with_thermal_model/LConn1 -- three_phase_inverter_mosfet_based_with_thermal_model/LConn1

== system single_phase_ttype_inverter/afe/brake ==
  Constant1 : Constant  Value=hwdata.afe.udc_nom
  Current Sensor3 : fl_lib/Electrical/Electrical Sensors/Current Sensor
  Integrator : Integrator
  MATLAB Function : MATLAB Function  TreatAsAtomicUnit=on  SystemSampleTime=glb_time.ts_afe
  PS-Simulink Converter : nesl_utility/PS-Simulink Converter  PhysicalDomain=network_engine_domain  SubClassName=ps_output  LeftPortType=input  RightPortType=output  PseudoPeriodic=off  Frequencies=[]  VectorFormat=1-D array  Unit=V  AffineConversion=off
  Product : Product
  Product6 : Product
  Rbrake : Subsystem
  Rbrake mod1 : Scope  NumInputPorts=2
      settings: SampleTime=glb_time.tc  ActiveDisplayYMinimum=-1  ActiveDisplayYMaximum=1  DataLoggingVariableName=ScopeData2
  Simulink-PS Converter4 : nesl_utility/Simulink-PS Converter  PhysicalDomain=network_engine_domain  SubClassName=ps_input  LeftPortType=input  RightPortType=output  PseudoPeriodic=off  Frequencies=[]  NoiseDistribution=none  NoiseParameters=[]  Unit=1  AffineConversion=on  FilteringAndDerivatives=provide  SimscapeFilterOrder=1  InputFilterTimeConstant=0.001  UdotUserProvided=0
  Step : Step  Time=time_aux_power_supply_fault  InitialValue=1  FinalValue=0  SampleTime=0
  To Workspace1 : ToWorkspace  VariableName=energy_Rbrake_sim_mod1  SampleTime=glb_time.tc
      settings: MaxDataPoints=glb_time.Nc
  To Workspace10 : ToWorkspace  VariableName=power_Rbrake_sim_mod1  SampleTime=glb_time.tc
      settings: MaxDataPoints=glb_time.Nc
  Unit Delay : UnitDelay  SampleTime=glb_time.ts_afe
  Voltage Sensor : fl_lib/Electrical/Electrical Sensors/Voltage Sensor
  Voltage Sensor1 : fl_lib/Electrical/Electrical Sensors/Voltage Sensor
  ibrakeR : nesl_utility/PS-Simulink Converter  PhysicalDomain=network_engine_domain  SubClassName=ps_output  LeftPortType=input  RightPortType=output  PseudoPeriodic=off  Frequencies=[]  VectorFormat=1-D array  Unit=A  AffineConversion=off
  switch_1 : Subsystem
      settings: PortSchema="{\"entries\":[{\"content\":{\"sides\":[{\"content\":{},\"type\":\"ConnectorPlacement.EquallySpacedRectSide\",\"uuid\":\"9277da8d-d460-43e6-8478-dd662f15d226\"},{\"content\":{\"side\":\"RIGHT\"},\"type\":\"ConnectorPlacement.EquallySpacedRectSide\",\"uuid\":\"a7ece396-f1d9-4f4f-a05b-db1fc65d6e1d\"},{\"content\":{\"connectorIds\":[\"LConn1\"],\"side\":\"TOP\"},\"type\":\"ConnectorPlacement.EquallySpacedRectSide\",\"uuid\":\"fdd70777-e9cf-4317-afb6-cae87f75d5b0\"},{\"content\":{\"connectorIds\":[\"RConn1\"],\"side\":\"BOTTOM\"},\"type\":\"ConnectorPlacement.EquallySpacedRectSide\",\"uuid\":\"2353ed68-b1a1-4775-9ca9-31e268d5443b\"}]},\"type\":\"ConnectorPlacement.EquallySpacedConnector\",\"uuid\":\"d5479f4c-4e65-4791-adcb-73df11f88590\"}],\"packageUris\":[\"http://schema.mathworks.com/mf0/Connector/R2020b\"],\"version\":\"1.0\"}"
  switch_2 : Subsystem
      settings: PortSchema="{\"entries\":[{\"content\":{\"sides\":[{\"content\":{\"connectorIds\":[\"LConn1\"]},\"type\":\"ConnectorPlacement.EquallySpacedRectSide\",\"uuid\":\"9277da8d-d460-43e6-8478-dd662f15d226\"},{\"content\":{\"connectorIds\":[],\"side\":\"RIGHT\"},\"type\":\"ConnectorPlacement.EquallySpacedRectSide\",\"uuid\":\"a7ece396-f1d9-4f4f-a05b-db1fc65d6e1d\"},{\"content\":{\"connectorIds\":[\"LConn2\"],\"side\":\"TOP\"},\"type\":\"ConnectorPlacement.EquallySpacedRectSide\",\"uuid\":\"fdd70777-e9cf-4317-afb6-cae87f75d5b0\"},{\"content\":{\"connectorIds\":[\"RConn1\"],\"side\":\"BOTTOM\"},\"type\":\"ConnectorPlacement.EquallySpacedRectSide\",\"uuid\":\"2353ed68-b1a1-4775-9ca9-31e268d5443b\"}]},\"type\":\"ConnectorPlacement.EquallySpacedConnector\",\"uuid\":\"d5479f4c-4e65-4791-adcb-73df11f88590\"}],\"packageUris\":[\"http://schema.mathworks.com/mf0/Connector/R2020b\"],\"version\":\"1.0\"}"
  ubrakeR : nesl_utility/PS-Simulink Converter  PhysicalDomain=network_engine_domain  SubClassName=ps_output  LeftPortType=input  RightPortType=output  PseudoPeriodic=off  Frequencies=[]  VectorFormat=1-D array  Unit=V  AffineConversion=off
  dc(+) : PMIOPort  Side=Left
  dc(-) : PMIOPort  Port=2  Side=Left
  tag scope: energy_Rbrake_mod1=global, power_Rbrake_mod1=global
  wires:
  Constant1/1 -> MATLAB Function/2(udc_ref)
  PS-Simulink Converter/1 -> MATLAB Function/1(u)
  MATLAB Function/1(y) -> Unit Delay/1
  ibrakeR/1 -> Product/1  "ibrakeR"
  ubrakeR/1 -> Product/2  "ubrakeR"
  Product/1 -> [power_Rbrake_mod1], Integrator/1
  Integrator/1 -> [energy_Rbrake_mod1]
  [power_Rbrake_mod1] -> To Workspace10/1, Rbrake mod1/1  "power_Rbrake"
  [energy_Rbrake_mod1] -> To Workspace1/1, Rbrake mod1/2  "energy_Rbrake"
  Step/1 -> Product6/1
  Unit Delay/1 -> Product6/2
  Product6/1 -> Simulink-PS Converter4/1
  connections:
  dc(-)/RConn1 -- switch_2/RConn1 -- Voltage Sensor/RConn2
  Voltage Sensor1/RConn2 -- Rbrake/RConn1 -- switch_1/RConn1 -- switch_2/LConn2
  PS-Simulink Converter/LConn1 -- Voltage Sensor/RConn1
  switch_2/LConn1 -- Simulink-PS Converter4/RConn1
  Voltage Sensor/LConn1 -- Current Sensor3/LConn1 -- switch_1/LConn1 -- dc(+)/RConn1
  Current Sensor3/RConn1 -- ibrakeR/LConn1
  Voltage Sensor1/RConn1 -- ubrakeR/LConn1
  Current Sensor3/RConn2 -- Voltage Sensor1/LConn1 -- Rbrake/LConn1

== system single_phase_ttype_inverter/battery_1/single_phase_ui_measure ==
  Bus Creator : BusCreator  Inputs=2
  Current Sensor : fl_lib/Electrical/Electrical Sensors/Current Sensor
  Selector : Selector  InputPortWidth=2  IndexOptions=Index vector (dialog)  Indices=2  OutputSizes=1
  Selector1 : Selector  InputPortWidth=2  IndexOptions=Index vector (dialog)  Indices=1  OutputSizes=1
  Terminator : Terminator
  Terminator1 : Terminator
  Voltage Sensor : fl_lib/Electrical/Electrical Sensors/Voltage Sensor
  dab input modA : Scope  NumInputPorts=2
      settings: SampleTime=glb_time.tc  ActiveDisplayYMinimum=1239.6508899029441  ActiveDisplayYMaximum=1249.6536701415532  DataLoggingVariableName=ScopeData2
  iph : nesl_utility/PS-Simulink Converter  PhysicalDomain=network_engine_domain  SubClassName=ps_output  LeftPortType=input  RightPortType=output  PseudoPeriodic=off  Frequencies=[]  VectorFormat=1-D array  Unit=A  AffineConversion=off
  uph : nesl_utility/PS-Simulink Converter  PhysicalDomain=network_engine_domain  SubClassName=ps_output  LeftPortType=input  RightPortType=output  PseudoPeriodic=off  Frequencies=[]  VectorFormat=1-D array  Unit=V  AffineConversion=off
  Udc(+) : PMIOPort  Side=Left
  udc(+) : PMIOPort  Port=2  Side=Right
  Udc(-) : PMIOPort  Port=3  Side=Left
  udc(-) : PMIOPort  Port=4  Side=Right
  tag scope: current_battery_1=global, voltage_battery_1=global
  wires:
  Bus Creator/1 -> Selector/1, Selector1/1  "ui_data"
  iph/1 -> Bus Creator/1  "iph"
  uph/1 -> Bus Creator/2  "uph"
  Selector1/1 -> [current_battery_1], dab input modA/1  "current_battery"
  Selector/1 -> dab input modA/2, [voltage_battery_1]  "voltage_battery"
  [current_battery_1] -> Terminator/1
  [voltage_battery_1] -> Terminator1/1
  connections:
  iph/LConn1 -- Current Sensor/RConn1
  Voltage Sensor/LConn1 -- Current Sensor/LConn1 -- Udc(+)/RConn1
  Current Sensor/RConn2 -- udc(+)/RConn1
  Voltage Sensor/RConn1 -- uph/LConn1
  Voltage Sensor/RConn2 -- Udc(-)/RConn1 -- udc(-)/RConn1

== system single_phase_ttype_inverter/dclink/references ==
  m : Inport
  Bus Selector : BusSelector  OutputSignals=udc,udc_p_gnd,udc_n_gnd,Cdc1_current
  Bus Selector1 : BusSelector  OutputSignals=idc1,idc2
  Bus Selector2 : BusSelector  OutputSignals=udc1,udc2
  tag scope: CFi_dc_current=global, dclink_n2gnd_voltage=global, dclink_p2gnd_voltage=global, dclink_voltage=global, idc1_m=global, idc2_m=global, udc1_m=global, udc2_m=global
  wires:
  Bus Selector1/1 -> [idc1_m]  "<idc1>"
  Bus Selector/1 -> [dclink_voltage]  "<udc>"
  Bus Selector/4 -> [CFi_dc_current]  "<Cdc1_current>"
  Bus Selector/3 -> [dclink_n2gnd_voltage]  "<udc_n_gnd>"
  Bus Selector/2 -> [dclink_p2gnd_voltage]  "<udc_p_gnd>"
  Bus Selector1/2 -> [idc2_m]  "<idc2>"
  m/1 -> Bus Selector/1, Bus Selector2/1, Bus Selector1/1
  Bus Selector2/1 -> [udc1_m]  "<udc1>"
  Bus Selector2/2 -> [udc2_m]  "<udc2>"

== system single_phase_ttype_inverter/global timing/time_afe1 ==
  correction_time : Inport
  Constant : Constant
  Gain : Gain  Gain=k
  Product : Product
  Sum : Sum  Inputs=|++
  time_1 : Clock
  Out1 : Outport
  wires:
  time_1/1 -> Gain/1
  Gain/1 -> Product/1
  Product/1 -> Out1/1
  correction_time/1 -> Sum/1
  Sum/1 -> Product/2
  Constant/1 -> Sum/2

== system single_phase_ttype_inverter/global timing/time_afe2 ==
  correction_time : Inport
  Constant : Constant
  Gain : Gain  Gain=k
  Product : Product
  Sum : Sum  Inputs=|++
  time_1 : Clock
  Out1 : Outport
  wires:
  Constant/1 -> Sum/2
  Sum/1 -> Product/2
  correction_time/1 -> Sum/1
  Product/1 -> Out1/1
  Gain/1 -> Product/1
  time_1/1 -> Gain/1

== system single_phase_ttype_inverter/global timing/time_afe3 ==
  Gain : Gain  Gain=k
  time_1 : Clock
  Out1 : Outport
  wires:
  Gain/1 -> Out1/1
  time_1/1 -> Gain/1

== system single_phase_ttype_inverter/grid/grid_emulator ==
  3ph_Dyg : Subsystem
  Bus Selector : BusSelector  OutputSignals=ua_grid_emu,ub_grid_emu,uc_grid_emu
  Bus Selector1 : BusSelector  OutputSignals=gamma_grid_emulator,omega_grid_emulator
  Controlled Voltage Source : fl_lib/Electrical/Electrical Sources/Controlled Voltage Source
  Controlled Voltage Source1 : fl_lib/Electrical/Electrical Sources/Controlled Voltage Source
  Controlled Voltage Source2 : fl_lib/Electrical/Electrical Sources/Controlled Voltage Source
  Electrical Reference : fl_lib/Electrical/Electrical Elements/Electrical Reference
  Simulink-PS Converter : nesl_utility/Simulink-PS Converter  PhysicalDomain=network_engine_domain  SubClassName=ps_input  LeftPortType=input  RightPortType=output  PseudoPeriodic=off  Frequencies=[]  NoiseDistribution=none  NoiseParameters=[]  Unit=V  AffineConversion=on  FilteringAndDerivatives=provide  SimscapeFilterOrder=1  InputFilterTimeConstant=0.001  UdotUserProvided=0
  Simulink-PS Converter1 : nesl_utility/Simulink-PS Converter  PhysicalDomain=network_engine_domain  SubClassName=ps_input  LeftPortType=input  RightPortType=output  PseudoPeriodic=off  Frequencies=[]  NoiseDistribution=none  NoiseParameters=[]  Unit=V  AffineConversion=on  FilteringAndDerivatives=provide  SimscapeFilterOrder=1  InputFilterTimeConstant=0.001  UdotUserProvided=0
  Simulink-PS Converter2 : nesl_utility/Simulink-PS Converter  PhysicalDomain=network_engine_domain  SubClassName=ps_input  LeftPortType=input  RightPortType=output  PseudoPeriodic=off  Frequencies=[]  NoiseDistribution=none  NoiseParameters=[]  Unit=V  AffineConversion=on  FilteringAndDerivatives=provide  SimscapeFilterOrder=1  InputFilterTimeConstant=0.001  UdotUserProvided=0
  Solver Configuration : nesl_utility/Solver Configuration  PhysicalDomain=network_engine_domain  SubClassName=solver  LeftPortType=input  RightPortType=generic  Tones=[]  Harmonics=[]  SimulateNoise=off  Profile=off  UseLocalSampling=off  EnableSwitchedLinearOptims=on  FrequencyDomain=off  UseCCode=off  RelTol=0.001  AbsTol=0.001  MinStep=1e-09  ToWorkspace=off  RevertToSquareIcSolve=off  NumHomotopyIterations=100  PhasorMode=off  PhasorModeNumHarmonics=1  ConsistencySolver=NEWTON_FTOL  CanonicalOrdering=UNORDERED  OptimizeIntermediates=UNOPTIMIZED  IndexReductionMethod=DerivativeReplacement  DoDC=on  ResidualTolerance=1e-3  ConsistencyTolSource=GLOBAL  ConsistencyAbsTol=0.001  ConsistencyRelTol=0.001  ConsistencyTolFactor=0.001  UseLocalSolver=on  LocalSolverChoice=NE_BACKWARD_EULER_ADVANCER  ResolveIndetEquations=on  FunctionEvalNumThread=1  LocalSolverSampleTime=glb_time.tc  DoFixedCost=on  MaxNonlinIter=nonlinear_iterations  MaxModeIter=2  ComputeImpulses=off  ImpulseIterations=2  LinearAlgebra=auto  LinearAlgebraNumThread=0  EquationFormulation=NE_TIME_EF  DelaysMemoryBudget=1024  AutomaticFiltering=on  FilteringTimeConstant=0.001  PartitionStorageMethod=AS_NEEDED  PartitionMemoryBudget=1024  PartitionMethod=ROBUST  MultibodyUseLocalSolver=off  MultibodyLocalSolverChoice=ODE1  MultibodyLocalSolverSampleTime=0.001
  three_phase_voltage_source_with_frt_emulator : three_phase_voltage_with_frt_emulator/three_phase_voltage_source_with_frt_emulator  nominal_frequency_m=grid_emu.fgrid_nom  nominal_voltage_m=grid_emu.us_primary_nom  Vemu_ref_norm_m=grid_emu.Vemu_ref_norm  vp_xi_pu_m=grid_emu.up_xi_pu_ref  vp_eta_pu_m=grid_emu.up_eta_pu_ref  vn_xi_pu_m=grid_emu.un_xi_pu_ref  vn_eta_pu_m=grid_emu.un_eta_pu_ref  Am=filters.afe.SOF_50Hz.ss_c.A  Bm=filters.afe.SOF_50Hz.ss_c.B  Cm=filters.afe.SOF_50Hz.ss_c.C  enable_frt_1_m=frt_data.enable_frt_1  enable_frt_2_m=frt_data.enable_frt_2  start_time_LVRT_m=frt_data.start_time_LVRT  end_time_LVRT_m=frt_data.end_time_LVRT  deepPOSxi_m=frt_data.deepPOSxi  deepPOSeta_m=frt_data.deepPOSeta  deepNEGxi_m=frt_data.deepNEGxi  deepNEGeta_m=frt_data.deepNEGeta  Amplitude_U_m=frt_data.Amplitude_U  Amplitude_V_m=frt_data.Amplitude_V  Amplitude_W_m=frt_data.Amplitude_W  t_ramp_m=frt_data.t_ramp  Phase_shift_m=frt_data.Phase_shift
  threephase_vi_measures : Subsystem
  u1 : PMIOPort  Side=Right
  u2 : PMIOPort  Port=2  Side=Right
  u3 : PMIOPort  Port=3  Side=Right
  tag scope: gamma_grid_emulator=global, omega_grid_emulator=global
  wires:
  Bus Selector1/2 -> [omega_grid_emulator]  "<omega_grid_emulator>"
  Bus Selector1/1 -> [gamma_grid_emulator]  "<gamma_grid_emulator>"
  Bus Selector/2 -> Simulink-PS Converter1/1  "<ub_grid_emu>"
  Bus Selector/3 -> Simulink-PS Converter2/1  "<uc_grid_emu>"
  three_phase_voltage_source_with_frt_emulator/1 -> Bus Selector1/1, Bus Selector/1
  Bus Selector/1 -> Simulink-PS Converter/1  "<ua_grid_emu>"
  connections:
  Simulink-PS Converter/RConn1 -- Controlled Voltage Source/RConn1
  Simulink-PS Converter1/RConn1 -- Controlled Voltage Source1/RConn1
  Simulink-PS Converter2/RConn1 -- Controlled Voltage Source2/RConn1
  Controlled Voltage Source/RConn2 -- Controlled Voltage Source1/RConn2 -- Controlled Voltage Source2/RConn2 -- Electrical Reference/LConn1 -- Solver Configuration/RConn1
  3ph_Dyg/RConn1 -- u1/RConn1
  3ph_Dyg/RConn2 -- u2/RConn1
  3ph_Dyg/RConn3 -- u3/RConn1
  3ph_Dyg/LConn1 -- threephase_vi_measures/RConn1
  3ph_Dyg/LConn2 -- threephase_vi_measures/RConn2
  3ph_Dyg/LConn3 -- threephase_vi_measures/RConn3
  Controlled Voltage Source/LConn1 -- threephase_vi_measures/LConn1
  Controlled Voltage Source1/LConn1 -- threephase_vi_measures/LConn2
  Controlled Voltage Source2/LConn1 -- threephase_vi_measures/LConn3
